simulink model "Ex4_LS3"  (R2025a)
settings: Solver=VariableStepAuto  StartTime=0.0  StopTime=10.0  RelTol=1e-3
values from neighbouring files (symbols this model uses):
  Beff = [50 50 50]    [Ex4_LS3_code_letra_a.m]    (also in Ex4_LS3_code_letra_b.m)
  F = 5    [Ex4_LS3_code_letra_a.m]    (also in Ex4_LS3_code_letra_b.m)
  Jeff = [14 14 14]    [Ex4_LS3_code_letra_a.m]    (also in Ex4_LS3_code_letra_b.m)
  K = 2750    [Ex4_LS3_code_letra_a.m]    (also in Ex4_LS3_code_letra_b.m)
  Kd = [(2*wn*Jeff(1) - Beff(1))/K (2*wn*Jeff(2) - Beff(2))/K (2*wn*Jeff(3) - Beff(3))/K]    [Ex4_LS3_code_letra_a.m]    (also in Ex4_LS3_code_letra_b.m)
  Kp = [(Jeff(1)*wn*wn)/K (Jeff(2)*wn*wn)/K (Jeff(3)*wn*wn)/K]    [Ex4_LS3_code_letra_a.m]    (also in Ex4_LS3_code_letra_b.m)
  L = [0.5; 0.3]    [Ex4_LS3_code_letra_a.m]    (also in Ex4_LS3_code_letra_b.m)
  m = [4.6; 2.3; 1.0]    [Ex4_LS3_code_letra_a.m]    (also in Ex4_LS3_code_letra_b.m)
  N = 3    [Ex4_LS3_code_letra_a.m]    (also in Ex4_LS3_code_letra_b.m)
  r = 1/100    (= 0.01)    [Ex4_LS3_code_letra_a.m]    (also in Ex4_LS3_code_letra_b.m)
libraries: slpidlib x1
settings Model: Creator=gusta  LastModifiedBy=Gabriel Toledo

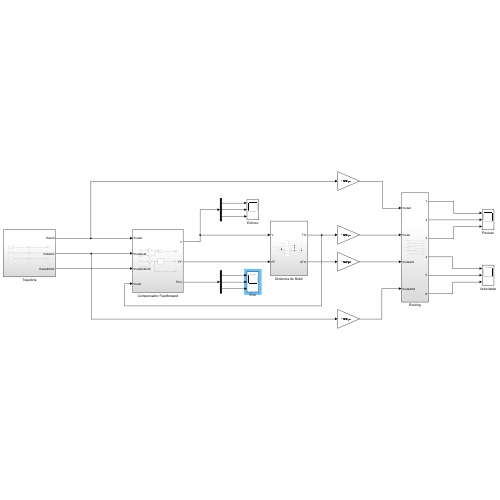
[thumbnail: Simulink's stored preview of the top-level diagram]
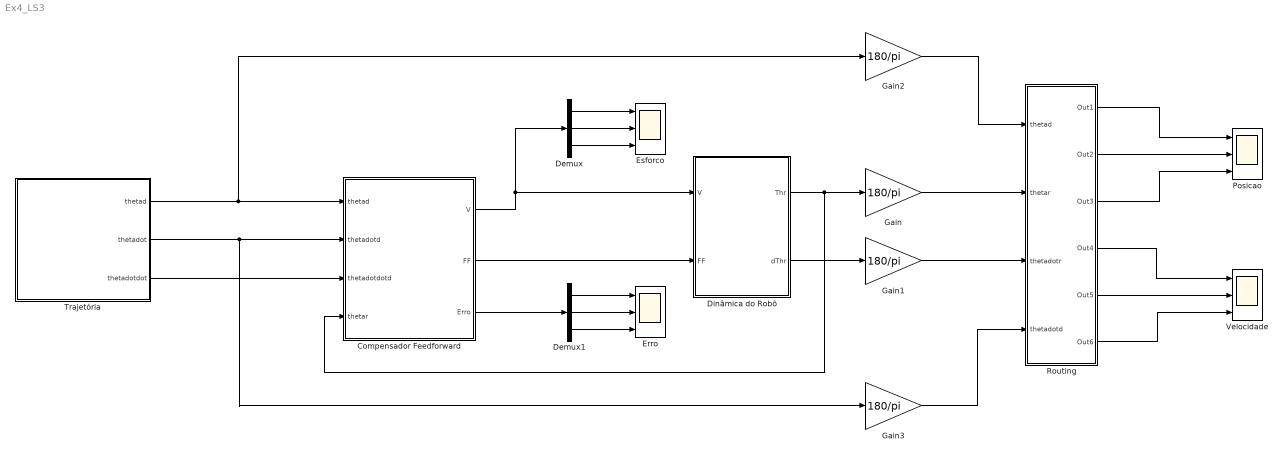
== system Ex4_LS3 ==
  Compensador Feedforward : Subsystem
  Demux : Demux  Outputs=3
  Demux1 : Demux  Outputs=3
  Dinâmica do Robô : Subsystem
  Erro : Scope  NumInputPorts=3
      settings: ActiveDisplayYMinimum=-0.0091697119544363326  ActiveDisplayYMaximum=0.15631954074254673  DataLoggingVariableName=Erro
  Esforco : Scope  NumInputPorts=3
      settings: ActiveDisplayYMinimum=-4861.2652  ActiveDisplayYMaximum=4798.38005  DataLoggingVariableName=Esforco
  Gain{,1..3} (4 alike) : Gain  Gain=180/pi
  Posicao : Scope  NumInputPorts=3
      settings: ActiveDisplayYMinimum=-260.38200695318278  ActiveDisplayYMaximum=161.18882096140891  DataLoggingVariableName=Posicao
  Routing : Subsystem
  Trajetória : Subsystem
  Velocidade : Scope  NumInputPorts=3
      settings: ActiveDisplayYMinimum=-110165.26508132949  ActiveDisplayYMaximum=105867.14567104682  DataLoggingVariableName=Velocidade
  wires:
  Compensador Feedforward/1(V) -> Demux/1, Dinâmica do Robô/1(V)
  Trajetória/1(thetad) -> Gain2/1, Compensador Feedforward/1(thetad)
  Trajetória/2(thetadot) -> Gain3/1, Compensador Feedforward/2(thetadotd)
  Trajetória/3(thetadotdot) -> Compensador Feedforward/3(thetadotdotd)
  Dinâmica do Robô/1(Thr) -> Gain/1, Compensador Feedforward/4(thetar)
  Dinâmica do Robô/2(dThr) -> Gain1/1
  Gain/1 -> Routing/2(thetar)
  Gain1/1 -> Routing/3(thetadotr)
  Demux/2 -> Esforco/2
  Demux/1 -> Esforco/1
  Demux/3 -> Esforco/3
  Demux1/1 -> Erro/1
  Demux1/2 -> Erro/2
  Demux1/3 -> Erro/3
  Compensador Feedforward/3(Erro) -> Demux1/1
  Routing/1(Out1) -> Posicao/1
  Routing/2(Out2) -> Posicao/2
  Routing/3(Out3) -> Posicao/3
  Routing/4(Out4) -> Velocidade/1
  Routing/5(Out5) -> Velocidade/2
  Routing/6(Out6) -> Velocidade/3
  Gain2/1 -> Routing/1(thetad)
  Gain3/1 -> Routing/4(thetadotd)
  Compensador Feedforward/2(FF) -> Dinâmica do Robô/2(FF)

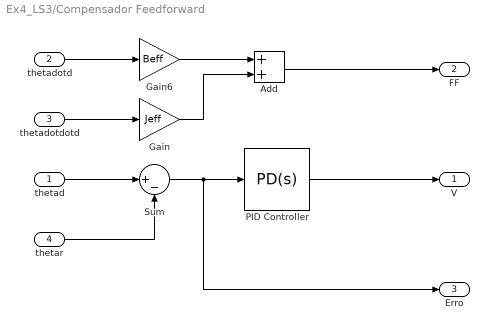
== system Ex4_LS3/Compensador Feedforward ==
  thetad : Inport
  thetadotd : Inport  Port=2
  thetadotdotd : Inport  Port=3
  thetar : Inport  Port=4
  Add : Sum
  Gain : Gain  Gain=Jeff
  Gain6 : Gain  Gain=Beff
  PID Controller : slpidlib/PID Controller  Controller=PD  Form=Parallel  TimeDomain=Continuous-time  UseExternalTs=off  SampleTime=-1  IntegratorMethod=Forward Euler  FilterMethod=Forward Euler  ControllerParametersSource=internal  P=Kp  I=1  UseKiTs=off  D=Kd  UseExternalDerivativeSource=off  N=N  UseFilter=on  TunerSelectOption=Transfer Function Based (PID Tuner App)  InitialConditionSource=internal  InitialConditionForIntegrator=0  InitialConditionForFilter=0  DifferentiatorICPrevScaledInput=0  ExternalReset=none  TrackingMode=off  Kt=1  LimitOutput=off  SatLimitsSource=internal  UpperSaturationLimit=inf  LowerSaturationLimit=-inf  LinearizeAsGain=on  AntiWindupMode=none  Kb=1  LimitIntegrator=off  UpperIntegratorSaturationLimit=inf  LowerIntegratorSaturationLimit=-inf  POutMin=[]  POutMax=[]  IOutMin=[]  IOutMax=[]  DOutMin=[]  DOutMax=[]  NOutMin=[]  NOutMax=[]  SumOutMin=[]  SumOutMax=[]  SaturationOutMin=[]  SaturationOutMax=[]  PParamMin=[]  PParamMax=[]  IParamMin=[]  IParamMax=[]  DParamMin=[]  DParamMax=[]  NParamMin=[]  NParamMax=[]  KbParamMin=[]  KbParamMax=[]  KtParamMin=[]  KtParamMax=[]  KbOutMin=[]  KbOutMax=[]  KtOutMin=[]  KtOutMax=[]  IntegratorOutMin=[]  IntegratorOutMax=[]  FilterOutMin=[]  FilterOutMax=[]  SumI1OutMin=[]  SumI1OutMax=[]  SumI2OutMin=[]  SumI2OutMax=[]  SumI3OutMin=[]  SumI3OutMax=[]  SumI4OutMin=[]  SumI4OutMax=[]  SumDOutMin=[]  SumDOutMax=[]  DifferentiatorOutMin=[]  DifferentiatorOutMax=[]  FilterDiffOutCoefMin=[]  FilterDiffOutCoefMax=[]  ReciprocalOutMin=[]  ReciprocalOutMax=[]  SumDenOutMin=[]  SumDenOutMax=[]  SumNumOutMin=[]  SumNumOutMax=[]  DivideOutMin=[]  DivideOutMax=[]  UdiffTsProdOutMin=[]  UdiffTsProdOutMax=[]  NTsProdOutMin=[]  NTsProdOutMax=[]  UintegralTsProdOutMin=[]  UintegralTsProdOutMax=[]  UngainTsProdOutMin=[]  UngainTsProdOutMax=[]  ClampingZeroOutDataTypeStr=Inherit: Inherit via back propagation  ClampingZeroOutMin=[]  ClampingZeroOutMax=[]  FilterDenConstantOutDataTypeStr=Inherit: Inherit via back propagation  FilterDenConstantOutMin=[]  FilterDenConstantOutMax=[]  PCopyOutDataTypeStr=Inherit: Inherit via back propagation  PCopyOutMin=[]  PCopyOutMax=[]  NCopyOutDataTypeStr=Inherit: Inherit via back propagation  NCopyOutMin=[]  NCopyOutMax=[]  IntegratorContinuousStateAttributes=''  IntegratorStateMustResolveToSignalObject=off  IntegratorRTWStateStorageClass=Auto  FilterContinuousStateAttributes=''  FilterStateMustResolveToSignalObject=off  FilterRTWStateStorageClass=Auto  ParallelPVariant=InternalParameters  IdealPVariant=Disabled  IVariant=Disabled  DVariant=InternalParameters  IntegratorVariant=Disabled  SatVariant=Disabled  AWVariant=Disabled  PCopyVariant=Disabled  TRVariant=Disabled  FdbkBlocksVariant=Forward  IdealPFdbkVariant=Disabled  SatFdbkVariant=Disabled  DerivativeFilterVariant=ContFilter  NVariant=InternalParameters  NCopyVariant=Disabled  FilterICVariant=InternalICsFilter  IntegratorICVariant=Disabled  ExternalResetVariant=Disabled  TRSumVariant=Passthrough  SumFdbkVariant=Disabled  SumVariant=Sum_PD  TsampFilterVariant=InternalTs  TsampNgainVariant=Passthrough  TsampIntegralVariant=Disabled_SignalSpec  ExternalSaturationOutDataTypeStr=Inherit: Same as second input  DerivativeSourceVariant=ErrorSignal  PreIntVariant=InternalPreInt
  Sum : Sum  Inputs=|+-
  V : Outport
  FF : Outport  Port=2
  Erro : Outport  Port=3
  wires:
  thetadotd/1 -> Gain6/1
  Gain6/1 -> Add/1
  Gain/1 -> Add/2
  thetadotdotd/1 -> Gain/1
  thetad/1 -> Sum/1
  thetar/1 -> Sum/2
  Sum/1 -> PID Controller/1, Erro/1
  Add/1 -> FF/1
  PID Controller/1 -> V/1

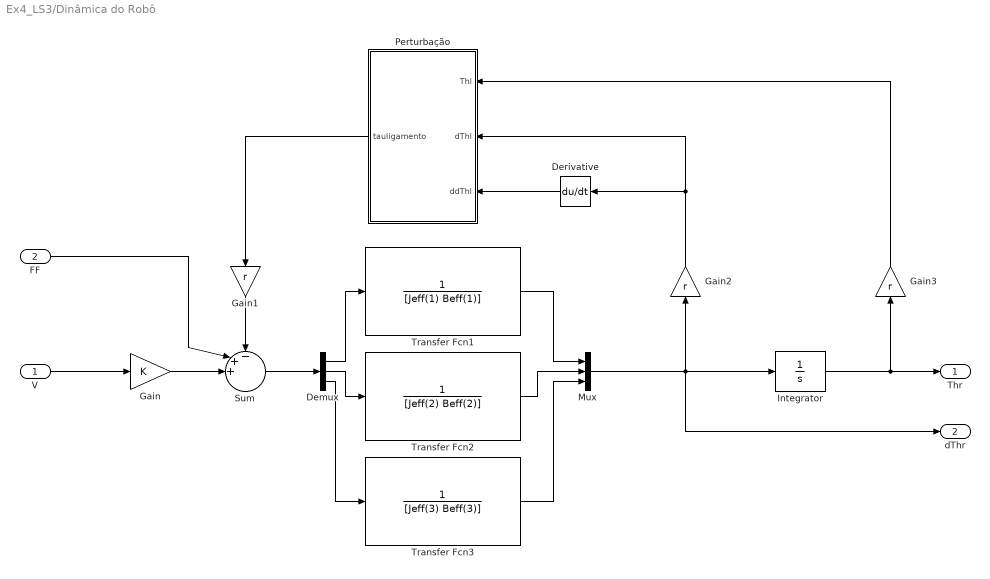
== system Ex4_LS3/Dinâmica do Robô ==
  V : Inport
  FF : Inport  Port=2
  Demux : Demux  Outputs=3
  Derivative : Derivative
  Gain : Gain  Gain=K
  Gain1 : Gain  Gain=r
  Gain2 : Gain  Gain=r
  Gain3 : Gain  Gain=r
  Integrator : Integrator
  Mux : Mux  Inputs=3
  Perturbação : Subsystem
  Sum : Sum  Inputs=-++||
  Transfer Fcn1 : TransferFcn  Denominator=[Jeff(1) Beff(1)]
  Transfer Fcn2 : TransferFcn  Denominator=[Jeff(2) Beff(2)]
  Transfer Fcn3 : TransferFcn  Denominator=[Jeff(3) Beff(3)]
  Thr : Outport
  dThr : Outport  Port=2
  wires:
  Integrator/1 -> Gain3/1, Thr/1
  Gain2/1 -> Perturbação/2(dThl), Derivative/1
  Derivative/1 -> Perturbação/3(ddThl)
  Perturbação/1(tauligamento) -> Gain1/1
  Gain3/1 -> Perturbação/1(Thl)
  V/1 -> Gain/1
  Gain1/1 -> Sum/1
  Gain/1 -> Sum/3
  FF/1 -> Sum/2
  Sum/1 -> Demux/1
  Demux/1 -> Transfer Fcn1/1
  Mux/1 -> dThr/1, Gain2/1, Integrator/1
  Transfer Fcn1/1 -> Mux/1
  Transfer Fcn3/1 -> Mux/3
  Transfer Fcn2/1 -> Mux/2
  Demux/2 -> Transfer Fcn2/1
  Demux/3 -> Transfer Fcn3/1

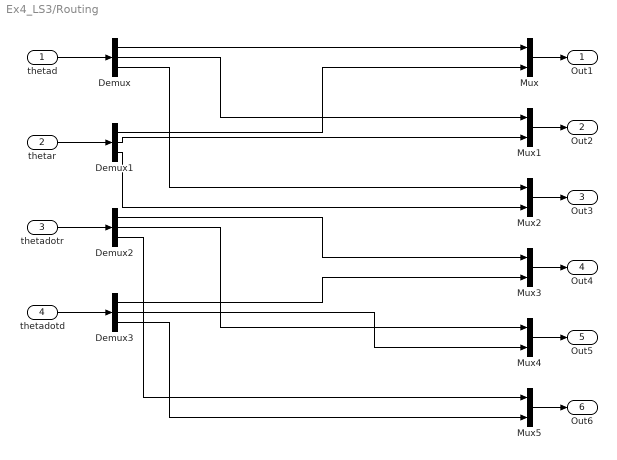
== system Ex4_LS3/Routing ==
  thetad : Inport
  thetar : Inport  Port=2
  thetadotr : Inport  Port=3
  thetadotd : Inport  Port=4
  Demux{,1..3} (4 alike) : Demux  Outputs=3
  Mux{,1..5} (6 alike) : Mux  Inputs=2
  Out1 : Outport
  Out2 : Outport  Port=2
  Out3 : Outport  Port=3
  Out4 : Outport  Port=4
  Out5 : Outport  Port=5
  Out6 : Outport  Port=6
  wires:
  thetad/1 -> Demux/1
  thetar/1 -> Demux1/1
  thetadotr/1 -> Demux2/1
  thetadotd/1 -> Demux3/1
  Demux/1 -> Mux/1
  Mux/1 -> Out1/1
  Mux2/1 -> Out3/1
  Mux1/1 -> Out2/1
  Mux3/1 -> Out4/1
  Mux5/1 -> Out6/1
  Mux4/1 -> Out5/1
  Demux1/1 -> Mux/2
  Demux/2 -> Mux1/1
  Demux1/2 -> Mux1/2
  Demux/3 -> Mux2/1
  Demux1/3 -> Mux2/2
  Demux2/1 -> Mux3/1
  Demux3/1 -> Mux3/2
  Demux2/2 -> Mux4/1
  Demux3/2 -> Mux4/2
  Demux3/3 -> Mux5/2
  Demux2/3 -> Mux5/1

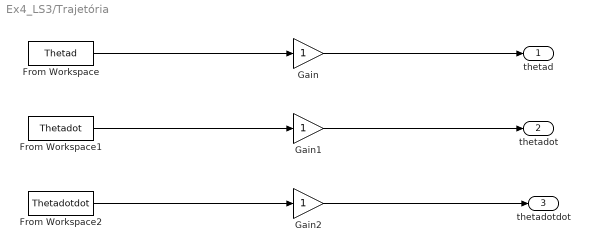
== system Ex4_LS3/Trajetória ==
  From Workspace : FromWorkspace  VariableName=Thetad
  From Workspace1 : FromWorkspace  VariableName=Thetadot
  From Workspace2 : FromWorkspace  VariableName=Thetadotdot
  Gain : Gain
  Gain1 : Gain
  Gain2 : Gain
  thetad : Outport
  thetadot : Outport  Port=2
  thetadotdot : Outport  Port=3
  wires:
  Gain/1 -> thetad/1
  From Workspace/1 -> Gain/1
  From Workspace1/1 -> Gain1/1
  Gain1/1 -> thetadot/1
  Gain2/1 -> thetadotdot/1
  From Workspace2/1 -> Gain2/1

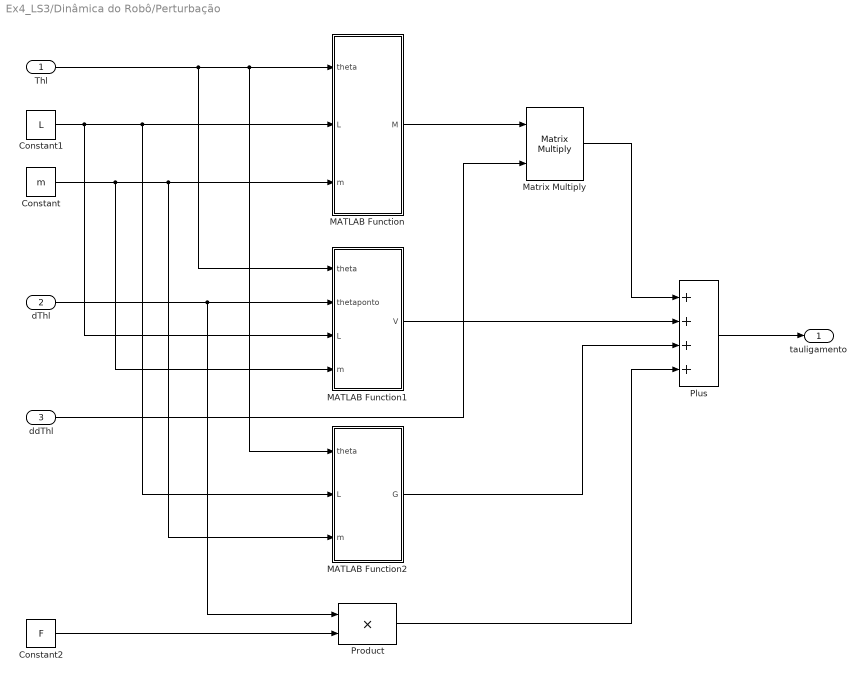
== system Ex4_LS3/Dinâmica do Robô/Perturbação ==
  Thl : Inport
  dThl : Inport  Port=2
  ddThl : Inport  Port=3
  Constant : Constant  Value=m
  Constant1 : Constant  Value=L
  Constant2 : Constant  Value=F
  MATLAB Function : MATLAB Function  TreatAsAtomicUnit=on
  MATLAB Function1 : MATLAB Function  TreatAsAtomicUnit=on
  MATLAB Function2 : MATLAB Function  TreatAsAtomicUnit=on
  Matrix Multiply : Product  Multiplication=Matrix(*)
  Plus : Sum  Inputs=++++
  Product : Product
  tauligamento : Outport
  wires:
  Constant/1 -> MATLAB Function1/4(m), MATLAB Function2/3(m), MATLAB Function/3(m)
  Constant1/1 -> MATLAB Function1/3(L), MATLAB Function2/2(L), MATLAB Function/2(L)
  Thl/1 -> MATLAB Function1/1(theta), MATLAB Function2/1(theta), MATLAB Function/1(theta)
  dThl/1 -> Product/1, MATLAB Function1/2(thetaponto)
  Plus/1 -> tauligamento/1
  MATLAB Function1/1(V) -> Plus/2
  MATLAB Function2/1(G) -> Plus/3
  Constant2/1 -> Product/2
  Product/1 -> Plus/4
  MATLAB Function/1(M) -> Matrix Multiply/1
  ddThl/1 -> Matrix Multiply/2
  Matrix Multiply/1 -> Plus/1

== matlab function Ex4_LS3/Dinâmica do Robô/Perturbação/MATLAB Function ==
  data: theta input; M output; L input; m input
function M = matriz_m(theta, L, m)

    M = [0,                                                 (m(2)+m(3))*(L(2)^2+L(1)*L(2))*cos(theta(3))+0.1,      0.1;
         (m(2)+m(3))*(L(2)^2+L(1)*L(2)*cos(theta(2)))+0.1,  0,                                                     0.1;
         0.1,                                               0.1,                                                   0];

== matlab function Ex4_LS3/Dinâmica do Robô/Perturbação/MATLAB Function1 ==
  data: theta input; thetaponto input; V output; L input; m input
function V = matriz_v(theta, thetaponto, L, m)
    
    V = [-(m(2)+m(3))*L(1)*L(2)*sin(theta(2))*(thetaponto(2)^2+thetaponto(1)*thetaponto(2));
         (m(2)+m(3))*L(1)*L(2)*sin(theta(2))*thetaponto(1)^2;
         0];

== matlab function Ex4_LS3/Dinâmica do Robô/Perturbação/MATLAB Function2 ==
  data: theta input; G output; L input; m input
function G = matriz_g(theta, L, m)
 
    G = [(m(1)+m(2)+m(3))*L(1)*cos(theta(1))+(m(2)+m(3))*(L(2)*cos(theta(1)+theta(2)));
         (m(2)+m(3))*(L(2)*cos(theta(1)+theta(2)));
         0];
